simulink model "LAB_3_SMNK"  (Simulink 7.4)
settings: Solver=ode1  SolverMode=SingleTasking  StartTime=0.0  StopTime=inf  FixedStep=T  RelTol=1e-3
undefined symbols (not defined in the file): Advantech, PCI, T
libraries: rtwinlib x2, simulink x2
settings Model: Creator=KG-MG  LastModifiedBy=MG  SimulationMode=external
settings OptimizationCC: InitFltsAndDblsToZero=on
settings DebuggingCC: SaveWithParameterizedLinksMsg=none  SignalResolutionControl=TryResolveAllWithWarning  MultiTaskDSMMsg=warning  MultiTaskCondExecSysMsg=none
settings RTWCC: SystemTargetFile=rtwin.tlc  TemplateMakefile=rtwin.tmf  Description=Real-Time Windows Target  ProcessScript=rtwin_make_rtw_hook  IncludeERTFirstTime=on
settings RTWinTargetCC: TargetFcnLib=ansi_tfl_tmw.mat  TargetLibSuffix=_rtwin.lib  TargetPreCompLibLocation=E:\Instalacje\Matlab2009b\toolbox\rtw\targets\rtwin\lib  TargetFunctionLibrary=ANSI_C  ModelReferenceCompliant=off  CompOptLevelCompliant=off  PortableWordSizes=off

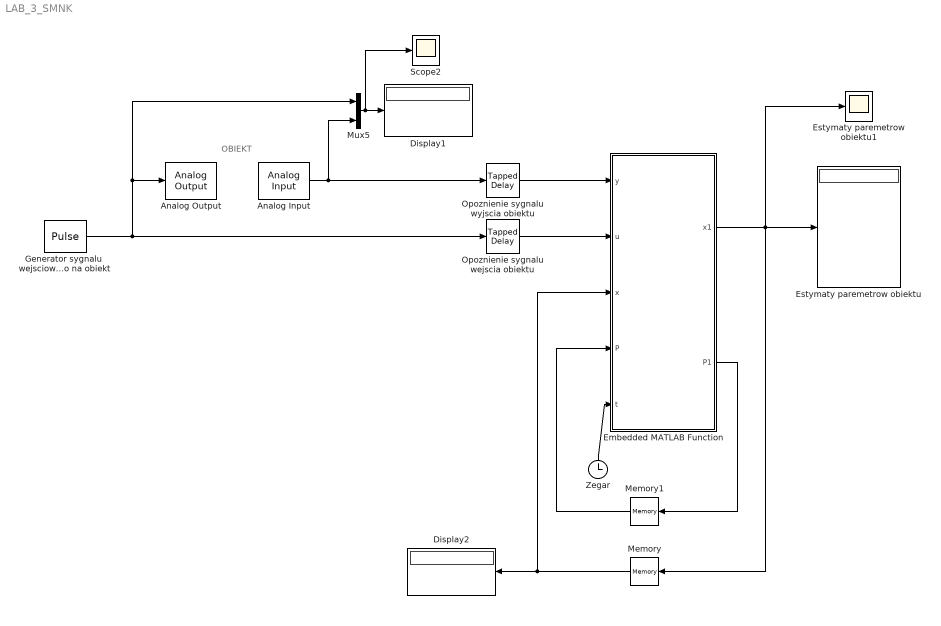
== system LAB_3_SMNK ==
  note: OBIEKT
  " Zegar" : Clock
  Analog Input : rtwinlib/Analog Input  SampleTime=T  DrvName=Advantech/PCI-1711  DrvAddress=4294967295  DrvOptions=zeros(1,0)  Channels=2  RangeMode=1  VoltRange=1  DataType=1
      settings: AttributesFormatString=Advantech\nPCI-1711 [auto]
  Analog Output : rtwinlib/Analog Output  SampleTime=T  DrvName=Advantech/PCI-1711  DrvAddress=4294967295  DrvOptions=zeros(1,0)  Channels=2  RangeMode=1  VoltRange=1  InitialValue=[]  FinalValue=[]
      settings: AttributesFormatString=Advantech\nPCI-1711 [auto]
  Display1 : Display
  Display2 : Display
  Embedded MATLAB Function : Stateflow chart  TreatAsAtomicUnit=on
  Estymaty paremetrow obiektu : Display
  Estymaty paremetrow obiektu1 : Scope
      settings: YMin=5.55112e-017  YMax=1
  Generator sygnalu  wejsciowego na obiekt : DiscretePulseGenerator  PulseType=Time based  Amplitude=1  Period=1  PulseWidth=50  PhaseDelay=0  SampleTime=1
  Memory : Memory
  Memory1 : Memory
  Mux5 : Mux  Inputs=2
  Opoznienie sygnalu wejscia obiektu : simulink/Discrete/Tapped Delay  vinit=0.0  samptime=T  NumDelays=1  DelayOrder=Oldest  includeCurrent=on
  Opoznienie sygnalu wyjscia obiektu : simulink/Discrete/Tapped Delay  vinit=0.0  samptime=T  NumDelays=1  DelayOrder=Oldest  includeCurrent=on
  Scope2 : Scope
      settings: YMin=0  YMax=1  SaveName=ScopeData2
  wires:
  Embedded MATLAB Function/1(x1) -> Estymaty paremetrow obiektu/1, Memory/1, Estymaty paremetrow obiektu1/1
  Memory/1 -> Display2/1, Embedded MATLAB Function/3(x)
  Opoznienie sygnalu wyjscia obiektu/1 -> Embedded MATLAB Function/1(y)
  Opoznienie sygnalu wejscia obiektu/1 -> Embedded MATLAB Function/2(u)
  " Zegar"/1 -> Embedded MATLAB Function/5(t)
  Embedded MATLAB Function/2(P1) -> Memory1/1
  Analog Input/1 -> Opoznienie sygnalu wyjscia obiektu/1, Mux5/2
  Generator sygnalu  wejsciowego na obiekt/1 -> Opoznienie sygnalu wejscia obiektu/1, Mux5/1, Analog Output/1
  Mux5/1 -> Display1/1, Scope2/1
  Memory1/1 -> Embedded MATLAB Function/4(P)

== matlab function Embedded MATLAB Function ==
  settings: fimath=|
      | fimath(...
      | 'RoundMode', 'floor',...
      | 'OverflowMode', 'wrap',...
      | 'ProductMode', 'KeepLSB', 'ProductWordLength', 32,...
      | 'SumMode', 'KeepLSB', 'SumWordLength', 32,...
      | 'CastBeforeSum', false)
  data: y input double; u input double; x1 output double; x input double; P input double; t input double; P1 output double
function [x1,P1]= fcn(y,u,x,P,t)
% This block supports an embeddable subset of the MATLAB language.
% See the help menu for details. 


% Parametry wejsciowe bloku
% y=wej(1:2);
% u=wej(3:4);
% x=wej(5:6);
% P=wej(7:10);
% t=wej(11);

%--------------------------------------------------------------------------
% parametry i inicjalizacja algorytmu
%--------------------------------------------------------------------------





%-------------------------------------------------------


if t==0     % Krok 0 - warunek poczatkowy
        H = ;                        
        W = ;                                        
        P1 = ;          
        x1 = ;

else t>0    % Krok kty >0

        H = 
        K = 
        P1 = 
        x1 = 
end
